simulink model "grasp_no_graphics"  (R2026a)
settings: Solver=daessc  StopTime=Run.timeout  MaxStep=0.001
undefined symbols (not defined in the file): C, km, Q, Run, U, X, Y, Z
libraries: sm_lib x80, nesl_utility x39, simulink x1
(part 1 of 3)
settings Model: Creator=kabir_09  LastModifiedBy=kabir_09
settings DebuggingCC: AlgebraicLoopMsg=error
settings SimscapeCC: SimscapeLogType=none
settings ExplorerConfigSet: SimMechanicsOpenEditorOnUpdate=off

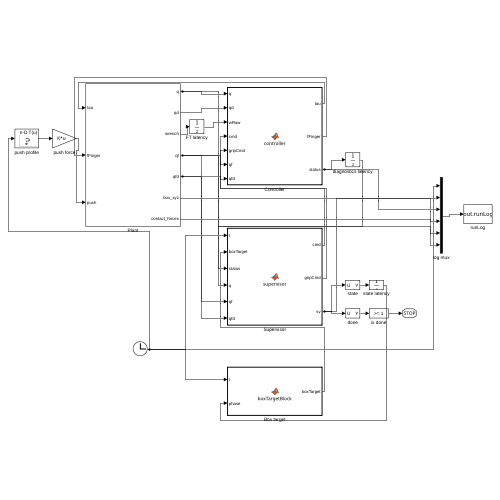
[thumbnail: Simulink's stored preview of the top-level diagram]
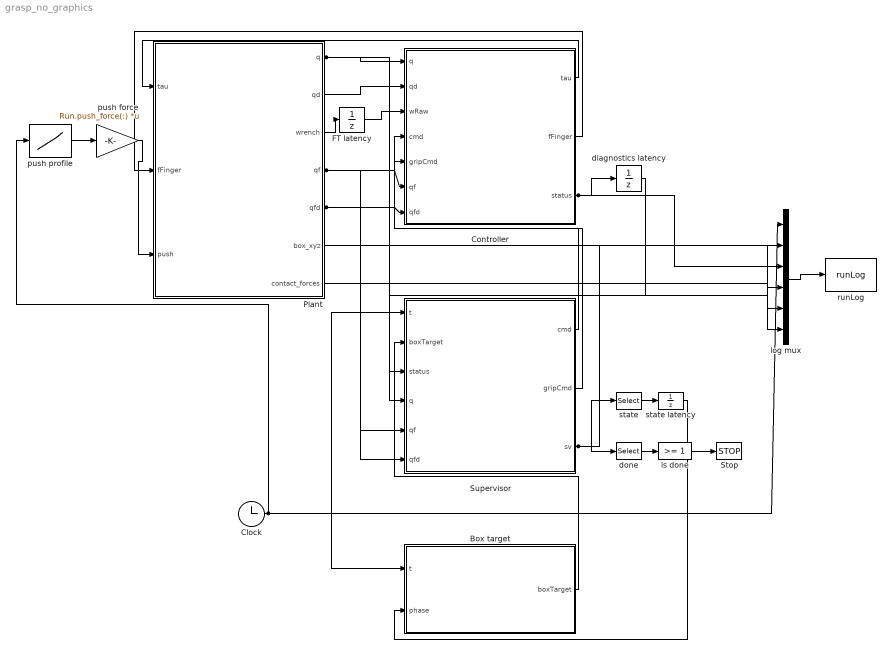
== system grasp_no_graphics ==
  Box target : MATLAB Function  TreatAsAtomicUnit=on  SystemSampleTime=0.02
  Clock : Clock
  Controller : MATLAB Function  TreatAsAtomicUnit=on  SystemSampleTime=0.001
  FT latency : UnitDelay  InitialCondition=zeros(6,1)  SampleTime=0.001
  Plant : Subsystem
  Stop : Stop
  Supervisor : MATLAB Function  TreatAsAtomicUnit=on  SystemSampleTime=0.02
  diagnostics latency : UnitDelay  InitialCondition=zeros(20,1)  SampleTime=0.001
  done : Selector  InputPortWidth=14  IndexOptions=Index vector (dialog)  Indices=4  OutputSizes=1
  is done : simulink/Logic and Bit Operations/Compare To Constant  relop=>=  const=1  OutDataTypeStr=boolean
  log mux : Mux  Inputs=6
  push force : Gain  Gain=Run.push_force(:)  Multiplication=Matrix(K*u)
  push profile : Lookup_n-D  NumberOfTableDimensions=1  BreakpointsForDimension1=Run.push_time  Table=Run.push_size  InternalRulePriority=Speed  RndMeth=Simplest
  runLog : ToWorkspace  VariableName=runLog  SampleTime=0.01
  state : Selector  InputPortWidth=14  IndexOptions=Index vector (dialog)  Indices=1  OutputSizes=1
  state latency : UnitDelay  SampleTime=0.02
  wires:
  Plant/1(q) -> Controller/1(q), Supervisor/4(q)
  Plant/2(qd) -> Controller/2(qd)
  Plant/3(wrench) -> FT latency/1
  FT latency/1 -> Controller/3(wRaw)
  Supervisor/1(cmd) -> Controller/4(cmd)
  Supervisor/2(gripCmd) -> Controller/5(gripCmd)
  Plant/4(qf) -> Controller/6(qf), Supervisor/5(qf), log mux/6
  Plant/5(qfd) -> Controller/7(qfd), Supervisor/6(qfd)
  Controller/1(tau) -> Plant/1(tau)
  Controller/2(fFinger) -> Plant/2(fFinger)
  Clock/1 -> push profile/1, Supervisor/1(t), Box target/1(t), log mux/1
  push profile/1 -> push force/1
  push force/1 -> Plant/3(push)
  Box target/1(boxTarget) -> Supervisor/2(boxTarget)
  Controller/3(status) -> diagnostics latency/1, log mux/3
  diagnostics latency/1 -> Supervisor/3(status)
  Supervisor/3(sv) -> state/1, done/1, log mux/2
  state/1 -> state latency/1
  state latency/1 -> Box target/2(phase)
  done/1 -> is done/1
  is done/1 -> Stop/1
  Plant/6(box_xyz) -> log mux/4
  Plant/7(contact_forces) -> log mux/5
  log mux/1 -> runLog/1
